simulink model "auto_sync_scan_module"  (R2016b)
settings: Solver=FixedStepDiscrete  StartTime=0.0  StopTime=3  FixedStep=Ts  RelTol=1e-3
InitFcn:
  | Ts = 50e-6;
values from neighbouring files (symbols this model uses):
  ScanStartTime = 0.2    [SISO_MIMO_blocks_Batch100_r2016b.m]
undefined symbols (not defined in the file or in its folder): freq
libraries: powerlib x17, powerlib_meascontrol x2
settings Model: Creator=rtlab17  LastModifiedBy=rtlab17

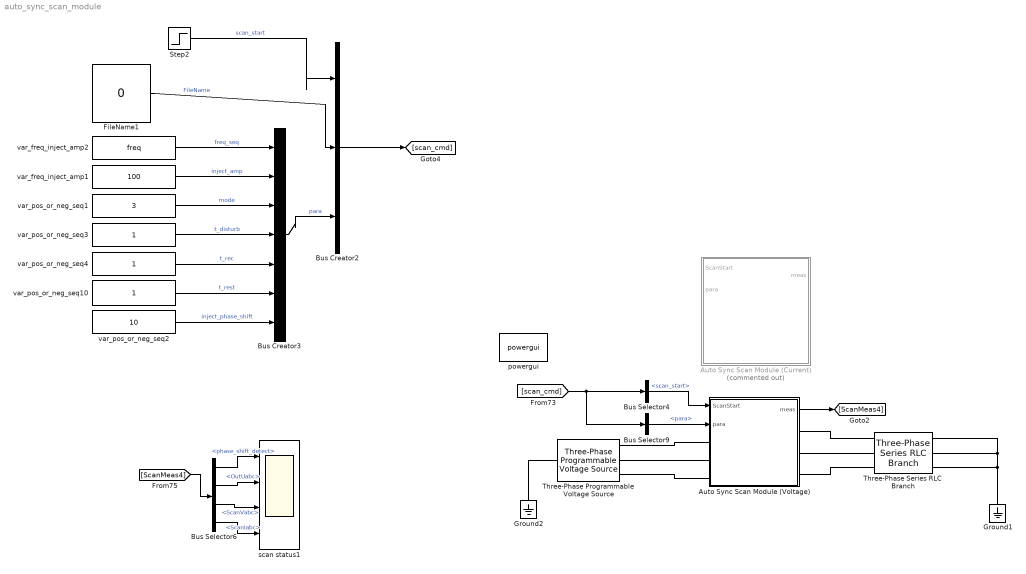
== system auto_sync_scan_module ==
  Auto Sync Scan Module (Current) : Subsystem  Commented=on  mask{var_gui_external=External, var_t_start=2, var_freq_seq=[1:350], var_inject_duration=1, var_record_duration=1, var_rest_duration=2, var_inject_amp=690*0.05, var_inject_mode=1, var_inject_phase_shift=0, var_ts=Ts}
      mask prompts: var_gui_external "Using"; var_t_start "Injection starting time (s)"; var_freq_seq "Frequency Sequence (Hz)"; var_inject_duration "Injection durtion (s)"; var_record_duration "Record duration (s), this set only output a recording signal"; var_rest_duration "Stable durtion (s)"; var_inject_amp "Injection magnitude. eg. 690*0.02"; var_inject_mode "Injection mode. eg 1 for Positive sequence, 2 for Negative, 3 for MIMO"; var_inject_phase_shift "Injection phase shift angle (deg). eg. if set 20 deg, disturb will injected when the phase angle 20deg of grid Uabc comes"; var_ts "Sample time"
      mask help:
      | |--------------Injection duration--------------|-----Stable duration------|
      |                      |-----Record duration-----|
      |
      | Record duration <= Inject duration
      |
      | Freq coupling implemented in this version
      mask init:
      | block = find_system(gcb,...
      |           'LookUnderMasks','on',...
      |           'FollowLinks','on','Name','In2');
      | % p=Simulink.Mask.get(gcb);
      | 
      | maskObj = Simulink.Mask.get(gcb);
      | [control, phandle] = maskObj.getDialogControl('para_group_gui_setting_zone');
      | 
      | switch var_gui_external
      |     case 1
      |         
      | %       if ~isempty(block)
      | % %         delete_block(block);
      | %         
      | %       end
      |       control.Visible = 'on';
      | 
      |       
      |       
      | %       p.getDialogControl('para_group_gui_setting_zone').Visible='on';
      |     case 2
      |         
      | %         if isempty(block)
      | % %             add_block('built-in/Inport',[gcb,'/In2']);
      | %         end
      |         
      |         control.Visible = 'off';
      | %         p.getDialogControl('para_group_gui_setting_zone').Visible='off';
      |     otherwise
      |         
      | end % switch
      | 
      | % disp(num2str(var_gui_external));
      mask Help:
      | by Yamin
      | v3(2024/11/28):
      | 1. fix: injection does not start when phase lag close to zero.
      | 2. refine the circuit connection topology.
      | 
      | v2(2024/5/17):
      | 1. add PLL phase alignment;
      | 2. Frequence sequence now can be specified by vector, elements could be random if you intend to do so.
      mask TypeOptions var_gui_external: GUI | External
      mask Display: text(0.3, 0.5, '电流源注入')
  Auto Sync Scan Module (Voltage) : Subsystem  mask{var_gui_external=External, var_t_start=2, var_freq_seq=[1:350], var_inject_duration=1, var_record_duration=1, var_rest_duration=2, var_inject_amp=690*0.05, var_inject_mode=1, var_inject_phase_shift=0, var_ts=Ts}
      mask prompts: var_gui_external "Using"; var_t_start "Injection starting time (s)"; var_freq_seq "Frequency Sequence (Hz)"; var_inject_duration "Injection durtion (s)"; var_record_duration "Record duration (s), this set only output a recording signal"; var_rest_duration "Stable durtion (s)"; var_inject_amp "Injection magnitude. eg. 690*0.02"; var_inject_mode "Injection mode. eg 1 for Positive sequence, 2 for Negative, 3 for MIMO"; var_inject_phase_shift "Injection phase shift angle (deg). eg. if set 20 deg, disturb will injected when the phase angle 20deg of grid Uabc comes"; var_ts "Sample time"
      mask help:
      | |--------------Injection duration--------------|-----Stable duration------|
      |                      |-----Record duration-----|
      |
      | Record duration <= Inject duration
      |
      | Freq coupling implemented in this version
      mask init: same as auto_sync_scan_module/Auto Sync Scan Module (Current)
      mask Help:
      | by Yamin
      | v3(2024/11/28):
      | 1. fix: injection does not start when phase lag close to zero.
      | 2. refine the circuit connection topology.
      | 
      | v2(2024/5/17):
      | 1. add PLL phase alignment;
      | 2. Frequence sequence now can be specified by vector, elements could be random if you intend to do so.
      mask TypeOptions var_gui_external: GUI | External
      mask Display: text(0.3, 0.5, '电压源注入')
  Bus Creator2 : BusCreator  Inputs=3
  Bus Creator3 : BusCreator  Inputs=7
  Bus Selector4 : BusSelector  OutputSignals=scan_start
  Bus Selector6 : BusSelector  OutputSignals=phase_shift_detect,OutUabc,ScanVabc,ScanIabc
  Bus Selector9 : BusSelector  OutputSignals=para
  FileName1 : Constant  Value=0
  Ground1 : powerlib/Elements/Ground  LConnTagsString=a
  Ground2 : powerlib/Elements/Ground  LConnTagsString=a
  Step2 : Step  Time=ScanStartTime  SampleTime=0
  Three-Phase Programmable Voltage Source : powerlib/Electrical Sources/Three-Phase Programmable Voltage Source  PositiveSequence="[230e3  0 50]"  VariationEntity=None  VariationType=Table of time-amplitude pairs  VariationTypeAlt=Step  VariationStep=0.5  VariationRate=10  VariationMagnitude=0.3  VariationFrequency=2  VariationTiming=[1 2]  VariationPhaseA=off  Amplitudes=[1 0.8 1.2 1.0]  TimeValues=[0 0.1 0.15 0.2]  HarmonicGeneration=off  HarmonicA=[3 0.2 -25 0]  HarmonicB=[2 0.15 35 2]  Timing="[0.05  3]"  BusType=PV  Pref=1100e6  Qref=0  Qmin=-inf  Qmax=inf
  Three-Phase Series RLC Branch : powerlib/Elements/Three-Phase Series RLC Branch  LConnTagsString=A|B|C  RConnTagsString=A|B|C  BranchType=RL  Resistance=1  Inductance=0.1  Capacitance=1e-6  Measurements=None
  powergui : powerlib/powergui  Priority=1  SimulationMode=Discrete  SolverType=Tustin/Backward Euler (TBE)  SampleTime=Ts  frequency=60  SPID=off  DisableSnubberDevices=off  DisableRonSwitches=off  DisableVfSwitches=off  SwTol=0  DisplayEquations=off  Interpol=off  ExternalGateDelay=off  methode=off  Ts=10  FunctionMessages=off  echomessages=off  HookPort=off  EnableUseOfTLC=off  x0status=blocks  frequencyindice=50  Pbase=100e6  ErrMax=1e-4  Iterations=50  UnitsV=kV  UnitsW=MW  buscounter=0  RestoreLinks=warning  ResistiveCurrentMeasurement=off  Frange=[0:2:500]  Ylog=off  Xlog=on  ShowGrid=off  save=off  variable=ZData  structure=0  ZoomFFT=off  StartTime=0.0  cycles=1  DisplayStyle=1  fundamental=60  FreqAxis=off  MaxFrequency=1000  frequencyindicesteady=1  RmsSteady=1  display=off
  scan status1 : Scope  NumInputPorts=4
  var_freq_inject_amp1 : Constant  Value=100
  var_freq_inject_amp2 : Constant  Value=freq
  var_pos_or_neg_seq1 : Constant  Value=3
  var_pos_or_neg_seq10 : Constant
  var_pos_or_neg_seq2 : Constant  Value=10
  var_pos_or_neg_seq3 : Constant
  var_pos_or_neg_seq4 : Constant
  wires:
  FileName1/1 -> Bus Creator2/2  "FileName"
  Step2/1 -> Bus Creator2/1  "scan_start"
  Bus Creator3/1 -> Bus Creator2/3  "para"
  var_freq_inject_amp1/1 -> Bus Creator3/2  "inject_amp"
  var_pos_or_neg_seq1/1 -> Bus Creator3/3  "mode"
  var_pos_or_neg_seq3/1 -> Bus Creator3/4  "t_disturb"
  var_pos_or_neg_seq4/1 -> Bus Creator3/5  "t_rec"
  var_pos_or_neg_seq10/1 -> Bus Creator3/6  "t_rest"
  var_freq_inject_amp2/1 -> Bus Creator3/1  "freq_seq"
  var_pos_or_neg_seq2/1 -> Bus Creator3/7  "inject_phase_shift"
  Bus Creator2/1 -> [scan_cmd]
  [ScanMeas4] -> Bus Selector6/1
  Bus Selector6/1 -> scan status1/1  "<phase_shift_detect>"
  Bus Selector6/2 -> scan status1/2  "<OutUabc>"
  Bus Selector4/1 -> Auto Sync Scan Module (Voltage)/1(ScanStart)  "<scan_start>"
  Bus Selector9/1 -> Auto Sync Scan Module (Voltage)/2(para)  "<para>"
  [scan_cmd] -> Bus Selector9/1, Bus Selector4/1
  Auto Sync Scan Module (Voltage)/1(meas) -> [ScanMeas4]
  Bus Selector6/3 -> scan status1/3  "<ScanVabc>"
  Bus Selector6/4 -> scan status1/4  "<ScanIabc>"
  connections:
  Ground2/LConn1 -- Three-Phase Programmable Voltage Source/LConn1
  Ground1/LConn1 -- Three-Phase Series RLC Branch/RConn3 -- Three-Phase Series RLC Branch/RConn1 -- Three-Phase Series RLC Branch/RConn2
  Auto Sync Scan Module (Voltage)/LConn2 -- Three-Phase Programmable Voltage Source/RConn2
  Auto Sync Scan Module (Voltage)/LConn3 -- Three-Phase Programmable Voltage Source/RConn3
  Auto Sync Scan Module (Voltage)/LConn1 -- Three-Phase Programmable Voltage Source/RConn1
  Auto Sync Scan Module (Voltage)/RConn1 -- Three-Phase Series RLC Branch/LConn1
  Auto Sync Scan Module (Voltage)/RConn2 -- Three-Phase Series RLC Branch/LConn2
  Auto Sync Scan Module (Voltage)/RConn3 -- Three-Phase Series RLC Branch/LConn3

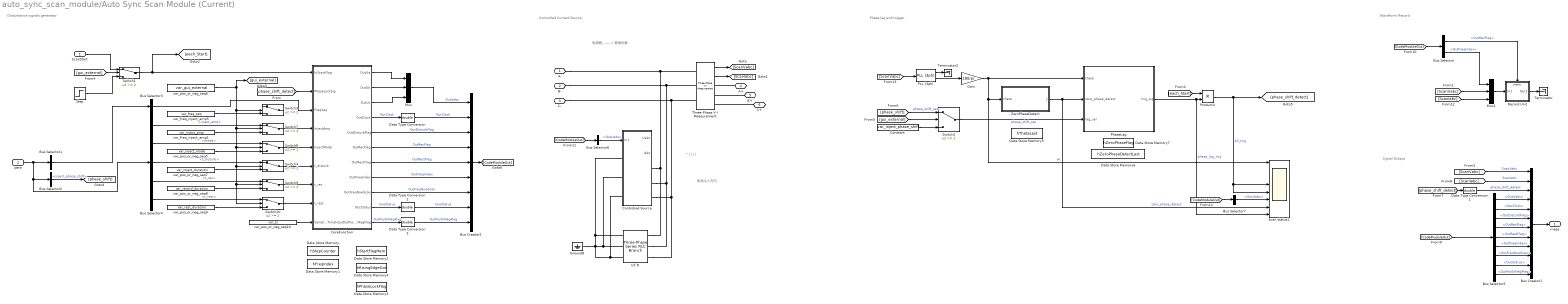
== system auto_sync_scan_module/Auto Sync Scan Module (Current) ==
  note: Disturbance signals generator
  note: Phase lag and trigger
  note: Waveform Record
  note: Signal Output
  note: 电流注入方向
  note: ^
      | |
      | |
      | |
      | |
  note: Controlled Current Source
  note: 电源侧 ------> 被测对象
  ScanStart : Inport
  para : Inport  Port=2
  Bus Creator1 : BusCreator  Inputs=12
  Bus Creator2 : BusCreator  Inputs=9
  Bus Selector : BusSelector  OutputSignals=OutRecFlag,OutFreqIndex
  Bus Selector1 : BusSelector  OutputSignals=freq_seq,inject_amp,mode,t_disturb,t_rec,t_rest  OutputAsBus=on
  Bus Selector2 : BusSelector  OutputSignals=inject_phase_shift
  Bus Selector3 : BusSelector  OutputSignals=freq_seq  OutputAsBus=on
  Bus Selector4 : BusSelector  OutputSignals=inject_amp,mode,t_disturb,t_rec,t_rest
  Bus Selector5 : BusSelector  OutputSignals=OutUabc,OutClock,OutDisturbFlag,OutRecFlag,OutRestFlag,OutFreqIndex,OutFreqNowScan,OutStatus,OutPosOrNegFlag
  Bus Selector6 : BusSelector  OutputSignals=OutUabc
  Bus Selector7 : BusSelector  OutputSignals=OutUabc
  Constant : Constant  Value=var_inject_phase_shift
  Controlled Source : Subsystem
  CoreFunction : MATLAB Function  TreatAsAtomicUnit=on  SystemSampleTime=var_ts
  Data Store Memory : DataStoreMemory  DataStoreName=hStepCounter  ReadBeforeWriteMsg=warning  WriteAfterWriteMsg=warning  WriteAfterReadMsg=warning  ShowAdditionalParam=off  OutDataTypeStr=int32
  Data Store Memory1 : DataStoreMemory  DataStoreName=hFreqIndex  ReadBeforeWriteMsg=warning  WriteAfterWriteMsg=warning  WriteAfterReadMsg=warning  ShowAdditionalParam=off  OutDataTypeStr=double
  Data Store Memory2 : DataStoreMemory  DataStoreName=hStartFlagMem  ReadBeforeWriteMsg=warning  WriteAfterWriteMsg=warning  WriteAfterReadMsg=warning  ShowAdditionalParam=off  OutDataTypeStr=int32
  Data Store Memory3 : DataStoreMemory  DataStoreName=hPhaseLockFlag  ReadBeforeWriteMsg=warning  WriteAfterWriteMsg=warning  WriteAfterReadMsg=warning  ShowAdditionalParam=off  OutDataTypeStr=double
  Data Store Memory4 : DataStoreMemory  DataStoreName=hRisingEdgeGot  ReadBeforeWriteMsg=warning  WriteAfterWriteMsg=warning  WriteAfterReadMsg=warning  ShowAdditionalParam=off  OutDataTypeStr=double
  Data Store Memory5 : DataStoreMemory  DataStoreName=hThetaLast  ReadBeforeWriteMsg=warning  WriteAfterWriteMsg=warning  WriteAfterReadMsg=warning  ShowAdditionalParam=off  OutDataTypeStr=double
  Data Store Memory6 : DataStoreMemory  DataStoreName=hZeroPhaseDetectLast  ReadBeforeWriteMsg=warning  WriteAfterWriteMsg=warning  WriteAfterReadMsg=warning  ShowAdditionalParam=off  OutDataTypeStr=double
  Data Store Memory7 : DataStoreMemory  DataStoreName=hZeroPhaseFlag  ReadBeforeWriteMsg=warning  WriteAfterWriteMsg=warning  WriteAfterReadMsg=warning  ShowAdditionalParam=off  OutDataTypeStr=double
  Data Type Conversion{,1..3} (4 alike) : DataTypeConversion  OutDataTypeStr=double
  Gain : Gain  Gain=180/pi
  Ground8 : powerlib/Elements/Ground  LConnTagsString=a
  Inf R : powerlib/Elements/Three-Phase Series RLC Branch  LConnTagsString=A|B|C  RConnTagsString=A|B|C  BranchType=R  Resistance=1e6  Inductance=4.57186*sin(deg2rad(85.2))/(100*pi)  Capacitance=1e-6  Measurements=None
  Mux : Mux  Inputs=3
  Mux1 : Mux  Inputs=3
  PLL (3ph) : powerlib_meascontrol/PLL/PLL (3ph)  Fmin=45  Par_Init=[0, 50]  ParK=[180, 3200, 1]  TcD=1e-4  MaxRateChangeFreq=12  FilterCutOffFreq=25  Ts=var_ts  AGC=on
  PhaseLag : MATLAB Function  TreatAsAtomicUnit=on
  Product4 : Product
  Record Unit : Subsystem
  Step : Step  Time=var_t_start  SampleTime=0
  Switch{1..2,4,7..10} (7 alike) : Switch  Threshold=2
  Switch3 : Switch  Threshold=2  AllowDiffInputSizes=on
  Terminator : Terminator
  Terminator2 : Terminator
  Three-Phase V-I Measurement : powerlib/Measurements/Three-Phase V-I Measurement  VoltageMeasurement=phase-to-ground  SetLabelV=off  LabelV=Vabc  Vpu=off  VpuLL=off  CurrentMeasurement=yes  SetLabelI=off  LabelI=Iabc  Ipu=off  Pbase=100e6  Vbase=500e3  OutputType=Complex  PhasorSimulation=off  PSBequivalent=0
  ZeroPhaseDetect : MATLAB Function  TreatAsAtomicUnit=on
  scan status1 : Scope  NumInputPorts=8
  var_freq_inject_amp1 : Constant  Value=var_inject_amp
  var_freq_inject_amp5 : Constant  Value=var_freq_seq
  var_pos_or_neg_seq10 : Constant  Value=var_ts
  var_pos_or_neg_seq5 : Constant  Value=var_inject_mode
  var_pos_or_neg_seq6 : Constant  Value=var_gui_external
  var_pos_or_neg_seq7 : Constant  Value=var_inject_duration
  var_pos_or_neg_seq8 : Constant  Value=var_record_duration
  var_pos_or_neg_seq9 : Constant  Value=var_rest_duration
  A- : PMIOPort  Port=1  Side=Left
  B- : PMIOPort  Port=2  Side=Left
  C- : PMIOPort  Port=3  Side=Left
  A+ : PMIOPort  Port=4  Side=Right
  B+ : PMIOPort  Port=5  Side=Right
  C+ : PMIOPort  Port=6  Side=Right
  meas : Outport
  wires:
  CoreFunction/9(OutFreqNowScan) -> Bus Creator2/7  "OutFreqNowScan"
  Bus Selector/1 -> Record Unit/Enable  "<OutRecFlag>"
  Bus Selector1/1 -> Bus Selector3/1
  var_pos_or_neg_seq10/1 -> CoreFunction/9(SampleTimeInput)
  var_pos_or_neg_seq6/1 -> Switch3/2, Switch7/2, Switch8/2, Switch4/2, Switch9/2, Switch10/2, [gui_external]
  CoreFunction/8(OutFreqIndex) -> Bus Creator2/6  "OutFreqIndex"
  CoreFunction/7(OutRestFlag) -> Bus Creator2/5  "OutRestFlag"
  CoreFunction/5(OutDisturbFlag) -> Bus Creator2/3  "OutDisturbFlag"
  CoreFunction/6(OutRecFlag) -> Bus Creator2/4  "OutRecFlag"
  Data Type Conversion2/1 -> Bus Creator2/8  "OutStatus"
  Data Type Conversion/1 -> Bus Creator2/2  "OutClock"
  Data Type Conversion3/1 -> Bus Creator2/9  "OutPosOrNegFlag"
  Mux/1 -> Bus Creator2/1  "OutUabc"
  CoreFunction/1(OutUa) -> Mux/1
  CoreFunction/3(OutUc) -> Mux/3
  CoreFunction/2(OutUb) -> Mux/2
  Switch7/1 -> CoreFunction/4(InjectAmp)
  Switch8/1 -> CoreFunction/5(InjectMode)
  Switch4/1 -> CoreFunction/6(t_disturb)
  Switch9/1 -> CoreFunction/7(t_rec)
  Switch10/1 -> CoreFunction/8(t_rest)
  var_pos_or_neg_seq9/1 -> Switch10/3
  var_pos_or_neg_seq8/1 -> Switch9/3
  var_pos_or_neg_seq7/1 -> Switch4/3
  var_pos_or_neg_seq5/1 -> Switch8/3
  var_freq_inject_amp1/1 -> Switch7/3
  var_freq_inject_amp5/1 -> Switch3/3
  Bus Selector4/1 -> Switch7/1  "<inject_amp>"
  Bus Selector4/4 -> Switch9/1  "<t_rec>"
  Bus Selector4/3 -> Switch4/1  "<t_disturb>"
  Bus Selector4/5 -> Switch10/1  "<t_rest>"
  Bus Selector4/2 -> Switch8/1  "<mode>"
  Bus Selector3/1 -> CoreFunction/3(FreqSeq)
  CoreFunction/11(OutPosOrNegFlag) -> Data Type Conversion3/1  "OutPosOrNegFlag"
  CoreFunction/10(OutStatus) -> Data Type Conversion2/1  "OutStatus"
  CoreFunction/4(OutClock) -> Data Type Conversion/1  "OutClock"
  Bus Selector/2 -> Mux1/1  "<OutFreqIndex>"
  Mux1/1 -> Record Unit/1(In1)
  Bus Creator2/1 -> [CodeModuleOut]
  PLL (3ph)/2 -> Gain/1
  Gain/1 -> scan status1/1, ZeroPhaseDetect/1(theta), PhaseLag/1(theta)  "wt"
  Constant/1 -> Switch2/3
  Product4/1 -> scan status1/5, scan status1/4, [phase_shift_detect]  "pll_trig"
  [each_Start] -> Product4/1
  Switch1/1 -> [each_Start], CoreFunction/1(InStartFlag)
  ScanStart/1 -> Switch1/1
  Step/1 -> Switch1/3
  Switch2/1 -> PhaseLag/3(lag_val)  "phase_shift_set"
  [gui_external] -> Switch2/2
  [gui_external] -> Switch1/2
  para/1 -> Bus Selector1/1, Bus Selector4/1, Bus Selector2/1
  Bus Selector2/1 -> [phase_shift]  "<inject_phase_shift>"
  [phase_shift] -> Switch2/1  "phase_shift_set"
  Bus Creator1/1 -> meas/1
  PLL (3ph)/1 -> Terminator2/1
  [phase_shift_detect] -> Data Type Conversion1/1
  Data Type Conversion1/1 -> Bus Creator1/3  "phase_shift_detect"
  [ScanVabc] -> Bus Creator1/1  "ScanVabc"
  [ScanIabc] -> Bus Creator1/2  "ScanIabc"
  Bus Selector5/3 -> Bus Creator1/6  "<OutDisturbFlag>"
  Bus Selector5/2 -> Bus Creator1/5  "<OutClock>"
  Bus Selector5/4 -> Bus Creator1/7  "<OutRecFlag>"
  Bus Selector5/1 -> Bus Creator1/4  "<OutUabc>"
  Bus Selector5/5 -> Bus Creator1/8  "<OutRestFlag>"
  Bus Selector5/6 -> Bus Creator1/9  "<OutFreqIndex>"
  Bus Selector5/7 -> Bus Creator1/10  "<OutFreqNowScan>"
  Bus Selector5/8 -> Bus Creator1/11  "<OutStatus>"
  Bus Selector5/9 -> Bus Creator1/12  "<OutPosOrNegFlag>"
  [CodeModuleOut] -> Bus Selector5/1
  Record Unit/1(Out1) -> Terminator/1
  [CodeModuleOut] -> Bus Selector/1
  ZeroPhaseDetect/1(y) -> scan status1/7, PhaseLag/2(zero_phase_detect)  "zero_phase_detect"
  PhaseLag/1(trig_sig) -> scan status1/8, Product4/2  "phase_lag_trig"
  [phase_shift_detect] -> CoreFunction/2(PhaseLockSig)
  [ScanVabc] -> Mux1/2
  [ScanIabc] -> Mux1/3
  [ScanVabc] -> PLL (3ph)/1
  [CodeModuleOut] -> Bus Selector7/1
  Bus Selector7/1 -> scan status1/6  "<OutUabc>"
  [CodeModuleOut] -> Bus Selector6/1
  Three-Phase V-I Measurement/2 -> [ScanIabc]
  Three-Phase V-I Measurement/1 -> [ScanVabc]
  Bus Selector6/1 -> Controlled Source/1(In1)  "<OutUabc>"
  connections:
  Controlled Source/RConn2 -- Inf R/LConn2 -- Three-Phase V-I Measurement/LConn2 -- B-/RConn1
  Inf R/LConn3 -- Controlled Source/RConn3 -- Three-Phase V-I Measurement/LConn3 -- C-/RConn1
  A-/RConn1 -- Three-Phase V-I Measurement/LConn1 -- Inf R/LConn1 -- Controlled Source/RConn1
  Controlled Source/LConn3 -- Inf R/RConn3 -- Ground8/LConn1 -- Inf R/RConn1 -- Controlled Source/LConn1 -- Inf R/RConn2 -- Controlled Source/LConn2
  C+/RConn1 -- Three-Phase V-I Measurement/RConn3
  B+/RConn1 -- Three-Phase V-I Measurement/RConn2
  A+/RConn1 -- Three-Phase V-I Measurement/RConn1

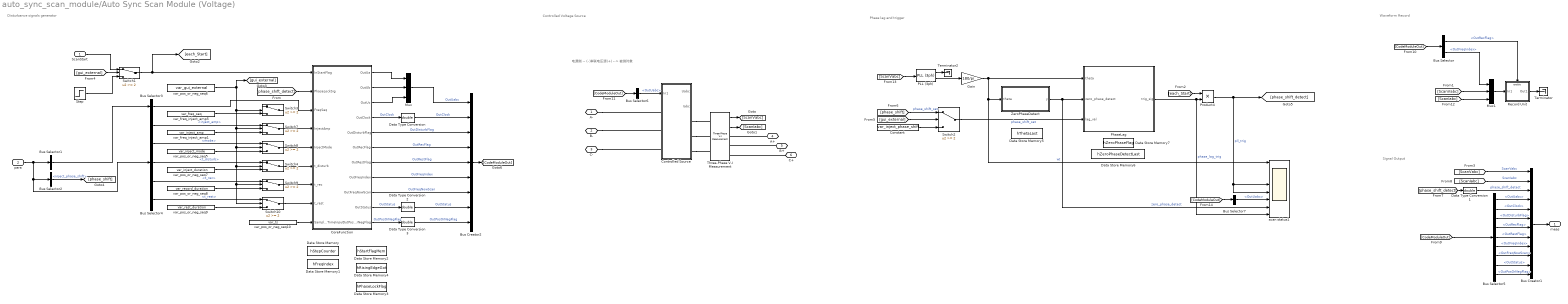
== system auto_sync_scan_module/Auto Sync Scan Module (Voltage) ==
  note: Signal Output
  note: Waveform Record
  note: Phase lag and trigger
  note: Disturbance signals generator
  note: Controlled Voltage Source
  note: 电源侧 -- (-)串联电压源(+) --> 被测对象
  ScanStart : Inport
  para : Inport  Port=2
  Bus Creator1 : BusCreator  Inputs=12
  Bus Creator2 : BusCreator  Inputs=9
  Bus Selector : BusSelector  OutputSignals=OutRecFlag,OutFreqIndex
  Bus Selector1 : BusSelector  OutputSignals=freq_seq,inject_amp,mode,t_disturb,t_rec,t_rest  OutputAsBus=on
  Bus Selector2 : BusSelector  OutputSignals=inject_phase_shift
  Bus Selector3 : BusSelector  OutputSignals=freq_seq  OutputAsBus=on
  Bus Selector4 : BusSelector  OutputSignals=inject_amp,mode,t_disturb,t_rec,t_rest
  Bus Selector5 : BusSelector  OutputSignals=OutUabc,OutClock,OutDisturbFlag,OutRecFlag,OutRestFlag,OutFreqIndex,OutFreqNowScan,OutStatus,OutPosOrNegFlag
  Bus Selector6 : BusSelector  OutputSignals=OutUabc
  Bus Selector7 : BusSelector  OutputSignals=OutUabc
  Constant : Constant  Value=var_inject_phase_shift
  Controlled Source : Subsystem
  CoreFunction : MATLAB Function  TreatAsAtomicUnit=on  SystemSampleTime=var_ts
  Data Store Memory : DataStoreMemory  DataStoreName=hStepCounter  ReadBeforeWriteMsg=warning  WriteAfterWriteMsg=warning  WriteAfterReadMsg=warning  ShowAdditionalParam=off  OutDataTypeStr=int32
  Data Store Memory1 : DataStoreMemory  DataStoreName=hFreqIndex  ReadBeforeWriteMsg=warning  WriteAfterWriteMsg=warning  WriteAfterReadMsg=warning  ShowAdditionalParam=off  OutDataTypeStr=double
  Data Store Memory2 : DataStoreMemory  DataStoreName=hStartFlagMem  ReadBeforeWriteMsg=warning  WriteAfterWriteMsg=warning  WriteAfterReadMsg=warning  ShowAdditionalParam=off  OutDataTypeStr=int32
  Data Store Memory3 : DataStoreMemory  DataStoreName=hPhaseLockFlag  ReadBeforeWriteMsg=warning  WriteAfterWriteMsg=warning  WriteAfterReadMsg=warning  ShowAdditionalParam=off  OutDataTypeStr=double
  Data Store Memory4 : DataStoreMemory  DataStoreName=hRisingEdgeGot  ReadBeforeWriteMsg=warning  WriteAfterWriteMsg=warning  WriteAfterReadMsg=warning  ShowAdditionalParam=off  OutDataTypeStr=double
  Data Store Memory5 : DataStoreMemory  DataStoreName=hThetaLast  ReadBeforeWriteMsg=warning  WriteAfterWriteMsg=warning  WriteAfterReadMsg=warning  ShowAdditionalParam=off  OutDataTypeStr=double
  Data Store Memory6 : DataStoreMemory  DataStoreName=hZeroPhaseDetectLast  ReadBeforeWriteMsg=warning  WriteAfterWriteMsg=warning  WriteAfterReadMsg=warning  ShowAdditionalParam=off  OutDataTypeStr=double
  Data Store Memory7 : DataStoreMemory  DataStoreName=hZeroPhaseFlag  ReadBeforeWriteMsg=warning  WriteAfterWriteMsg=warning  WriteAfterReadMsg=warning  ShowAdditionalParam=off  OutDataTypeStr=double
  Data Type Conversion{,1..3} (4 alike) : DataTypeConversion  OutDataTypeStr=double
  Gain : Gain  Gain=180/pi
  Mux : Mux  Inputs=3
  Mux1 : Mux  Inputs=3
  PLL (3ph) : powerlib_meascontrol/PLL/PLL (3ph)  Fmin=45  Par_Init=[0, 50]  ParK=[180, 3200, 1]  TcD=1e-4  MaxRateChangeFreq=12  FilterCutOffFreq=25  Ts=var_ts  AGC=on
  PhaseLag : MATLAB Function  TreatAsAtomicUnit=on
  Product4 : Product
  Record Unit : Subsystem
  Step : Step  Time=var_t_start  SampleTime=0
  Switch{1..2,4,7..10} (7 alike) : Switch  Threshold=2
  Switch3 : Switch  Threshold=2  AllowDiffInputSizes=on
  Terminator : Terminator
  Terminator2 : Terminator
  Three-Phase V-I Measurement : powerlib/Measurements/Three-Phase V-I Measurement  VoltageMeasurement=phase-to-ground  SetLabelV=off  LabelV=Vabc  Vpu=off  VpuLL=off  CurrentMeasurement=yes  SetLabelI=off  LabelI=Iabc  Ipu=off  Pbase=100e6  Vbase=500e3  OutputType=Complex  PhasorSimulation=off  PSBequivalent=0
  ZeroPhaseDetect : MATLAB Function  TreatAsAtomicUnit=on
  scan status1 : Scope  NumInputPorts=8
  var_freq_inject_amp1 : Constant  Value=var_inject_amp
  var_freq_inject_amp5 : Constant  Value=var_freq_seq
  var_pos_or_neg_seq10 : Constant  Value=var_ts
  var_pos_or_neg_seq5 : Constant  Value=var_inject_mode
  var_pos_or_neg_seq6 : Constant  Value=var_gui_external
  var_pos_or_neg_seq7 : Constant  Value=var_inject_duration
  var_pos_or_neg_seq8 : Constant  Value=var_record_duration
  var_pos_or_neg_seq9 : Constant  Value=var_rest_duration
  A- : PMIOPort  Port=1  Side=Left
  B- : PMIOPort  Port=2  Side=Left
  C- : PMIOPort  Port=3  Side=Left
  A+ : PMIOPort  Port=4  Side=Right
  B+ : PMIOPort  Port=5  Side=Right
  C+ : PMIOPort  Port=6  Side=Right
  meas : Outport
  wires:
  Bus Selector7/1 -> scan status1/6  "<OutUabc>"
  [CodeModuleOut] -> Bus Selector7/1
  [ScanVabc] -> PLL (3ph)/1
  [ScanIabc] -> Mux1/3
  [ScanVabc] -> Mux1/2
  [phase_shift_detect] -> CoreFunction/2(PhaseLockSig)
  PhaseLag/1(trig_sig) -> Product4/2, scan status1/8  "phase_lag_trig"
  ZeroPhaseDetect/1(y) -> PhaseLag/2(zero_phase_detect), scan status1/7  "zero_phase_detect"
  [CodeModuleOut] -> Bus Selector6/1
  [CodeModuleOut] -> Bus Selector/1
  Record Unit/1(Out1) -> Terminator/1
  [CodeModuleOut] -> Bus Selector5/1
  Bus Selector5/9 -> Bus Creator1/12  "<OutPosOrNegFlag>"
  Bus Selector5/8 -> Bus Creator1/11  "<OutStatus>"
  Bus Selector5/7 -> Bus Creator1/10  "<OutFreqNowScan>"
  Bus Selector5/6 -> Bus Creator1/9  "<OutFreqIndex>"
  Bus Selector5/5 -> Bus Creator1/8  "<OutRestFlag>"
  Bus Selector5/1 -> Bus Creator1/4  "<OutUabc>"
  Bus Selector5/4 -> Bus Creator1/7  "<OutRecFlag>"
  Bus Selector5/2 -> Bus Creator1/5  "<OutClock>"
  Bus Selector5/3 -> Bus Creator1/6  "<OutDisturbFlag>"
  [ScanIabc] -> Bus Creator1/2  "ScanIabc"
  [ScanVabc] -> Bus Creator1/1  "ScanVabc"
  Data Type Conversion1/1 -> Bus Creator1/3  "phase_shift_detect"
  [phase_shift_detect] -> Data Type Conversion1/1
  PLL (3ph)/1 -> Terminator2/1
  Bus Creator1/1 -> meas/1
  [phase_shift] -> Switch2/1  "phase_shift_set"
  Bus Selector2/1 -> [phase_shift]  "<inject_phase_shift>"
  para/1 -> Bus Selector2/1, Bus Selector4/1, Bus Selector1/1
  [gui_external] -> Switch1/2
  [gui_external] -> Switch2/2
  Switch2/1 -> PhaseLag/3(lag_val)  "phase_shift_set"
  Three-Phase V-I Measurement/2 -> [ScanIabc]
  Step/1 -> Switch1/3
  ScanStart/1 -> Switch1/1
  Switch1/1 -> CoreFunction/1(InStartFlag), [each_Start]
  [each_Start] -> Product4/1
  Product4/1 -> [phase_shift_detect], scan status1/4, scan status1/5  "pll_trig"
  Constant/1 -> Switch2/3
  Gain/1 -> PhaseLag/1(theta), ZeroPhaseDetect/1(theta), scan status1/1  "wt"
  PLL (3ph)/2 -> Gain/1
  Three-Phase V-I Measurement/1 -> [ScanVabc]
  Bus Creator2/1 -> [CodeModuleOut]
  Bus Selector6/1 -> Controlled Source/1(In1)  "<OutUabc>"
  Mux1/1 -> Record Unit/1(In1)
  Bus Selector/2 -> Mux1/1  "<OutFreqIndex>"
  CoreFunction/4(OutClock) -> Data Type Conversion/1  "OutClock"
  CoreFunction/10(OutStatus) -> Data Type Conversion2/1  "OutStatus"
  CoreFunction/11(OutPosOrNegFlag) -> Data Type Conversion3/1  "OutPosOrNegFlag"
  Bus Selector3/1 -> CoreFunction/3(FreqSeq)
  Bus Selector4/2 -> Switch8/1  "<mode>"
  Bus Selector4/5 -> Switch10/1  "<t_rest>"
  Bus Selector4/3 -> Switch4/1  "<t_disturb>"
  Bus Selector4/4 -> Switch9/1  "<t_rec>"
  Bus Selector4/1 -> Switch7/1  "<inject_amp>"
  var_freq_inject_amp5/1 -> Switch3/3
  var_freq_inject_amp1/1 -> Switch7/3
  var_pos_or_neg_seq5/1 -> Switch8/3
  var_pos_or_neg_seq7/1 -> Switch4/3
  var_pos_or_neg_seq8/1 -> Switch9/3
  var_pos_or_neg_seq9/1 -> Switch10/3
  Switch10/1 -> CoreFunction/8(t_rest)
  Switch9/1 -> CoreFunction/7(t_rec)
  Switch4/1 -> CoreFunction/6(t_disturb)
  Switch8/1 -> CoreFunction/5(InjectMode)
  Switch7/1 -> CoreFunction/4(InjectAmp)
  CoreFunction/2(OutUb) -> Mux/2
  CoreFunction/3(OutUc) -> Mux/3
  CoreFunction/1(OutUa) -> Mux/1
  Mux/1 -> Bus Creator2/1  "OutUabc"
  Data Type Conversion3/1 -> Bus Creator2/9  "OutPosOrNegFlag"
  Data Type Conversion/1 -> Bus Creator2/2  "OutClock"
  Data Type Conversion2/1 -> Bus Creator2/8  "OutStatus"
  CoreFunction/6(OutRecFlag) -> Bus Creator2/4  "OutRecFlag"
  CoreFunction/5(OutDisturbFlag) -> Bus Creator2/3  "OutDisturbFlag"
  CoreFunction/7(OutRestFlag) -> Bus Creator2/5  "OutRestFlag"
  CoreFunction/8(OutFreqIndex) -> Bus Creator2/6  "OutFreqIndex"
  var_pos_or_neg_seq6/1 -> [gui_external], Switch10/2, Switch9/2, Switch4/2, Switch8/2, Switch7/2, Switch3/2
  var_pos_or_neg_seq10/1 -> CoreFunction/9(SampleTimeInput)
  Bus Selector1/1 -> Bus Selector3/1
  Bus Selector/1 -> Record Unit/Enable  "<OutRecFlag>"
  CoreFunction/9(OutFreqNowScan) -> Bus Creator2/7  "OutFreqNowScan"
  connections:
  C+/RConn1 -- Three-Phase V-I Measurement/RConn3
  B+/RConn1 -- Three-Phase V-I Measurement/RConn2
  A+/RConn1 -- Three-Phase V-I Measurement/RConn1
  Controlled Source/RConn2 -- Three-Phase V-I Measurement/LConn2
  Controlled Source/RConn3 -- Three-Phase V-I Measurement/LConn3
  Controlled Source/RConn1 -- Three-Phase V-I Measurement/LConn1
  C-/RConn1 -- Controlled Source/LConn3
  B-/RConn1 -- Controlled Source/LConn2
  A-/RConn1 -- Controlled Source/LConn1

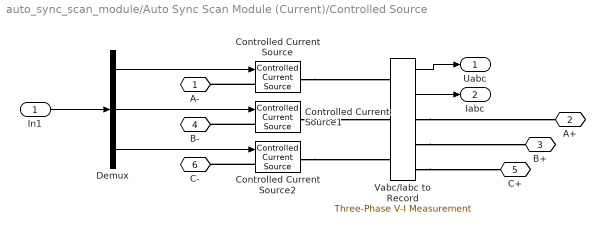
== system auto_sync_scan_module/Auto Sync Scan Module (Current)/Controlled Source ==
  In1 : Inport
  Controlled Current Source : powerlib/Electrical Sources/Controlled Current Source  Initialize=on  Source_Type=AC  Amplitude=0  Phase=0  Frequency=0  Measurements=None
  Controlled Current Source1 : powerlib/Electrical Sources/Controlled Current Source  Initialize=on  Source_Type=AC  Amplitude=0  Phase=0  Frequency=0  Measurements=None
  Controlled Current Source2 : powerlib/Electrical Sources/Controlled Current Source  Initialize=on  Source_Type=AC  Amplitude=0  Phase=0  Frequency=0  Measurements=None
  Demux : Demux  Outputs=3
  Vabc/Iabc to Record : powerlib/Measurements/Three-Phase V-I Measurement  VoltageMeasurement=phase-to-ground  SetLabelV=off  LabelV=ScanVabc  Vpu=off  VpuLL=off  CurrentMeasurement=yes  SetLabelI=off  LabelI=ScanIabc  Ipu=off  Pbase=100e6  Vbase=500e3  OutputType=Complex  PhasorSimulation=off  PSBequivalent=0
  A- : PMIOPort  Port=1  Side=Left
  A+ : PMIOPort  Port=2  Side=Right
  B+ : PMIOPort  Port=3  Side=Right
  B- : PMIOPort  Port=4  Side=Left
  C+ : PMIOPort  Port=5  Side=Right
  C- : PMIOPort  Port=6  Side=Left
  Uabc : Outport
  Iabc : Outport  Port=2
  wires:
  Demux/3 -> Controlled Current Source2/1
  Demux/2 -> Controlled Current Source1/1
  Demux/1 -> Controlled Current Source/1
  In1/1 -> Demux/1
  Vabc/Iabc to Record/1 -> Uabc/1
  Vabc/Iabc to Record/2 -> Iabc/1
  connections:
  Vabc/Iabc to Record/RConn1 -- A+/RConn1
  Controlled Current Source/RConn1 -- Vabc/Iabc to Record/LConn1
  Controlled Current Source1/RConn1 -- Vabc/Iabc to Record/LConn2
  Controlled Current Source2/RConn1 -- Vabc/Iabc to Record/LConn3
  Vabc/Iabc to Record/RConn3 -- C+/RConn1
  Controlled Current Source/LConn1 -- A-/RConn1
  Controlled Current Source1/LConn1 -- B-/RConn1
  Vabc/Iabc to Record/RConn2 -- B+/RConn1
  Controlled Current Source2/LConn1 -- C-/RConn1

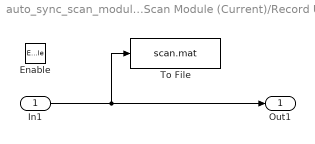
== system auto_sync_scan_module/Auto Sync Scan Module (Current)/Record Unit ==
  In1 : Inport
  Enable : EnablePort
  To File : ToFile  Filename=scan.mat  MatrixName=scan  SampleTime=var_ts
  Out1 : Outport
  wires:
  In1/1 -> Out1/1, To File/1

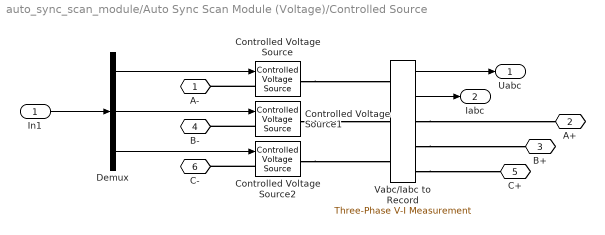
== system auto_sync_scan_module/Auto Sync Scan Module (Voltage)/Controlled Source ==
  In1 : Inport
  Controlled Voltage Source : powerlib/Electrical Sources/Controlled Voltage Source  Initialize=on  Source_Type=AC  Amplitude=0  Phase=0  Frequency=0  Measurements=None
  Controlled Voltage Source1 : powerlib/Electrical Sources/Controlled Voltage Source  Initialize=on  Source_Type=AC  Amplitude=0  Phase=0  Frequency=0  Measurements=None
  Controlled Voltage Source2 : powerlib/Electrical Sources/Controlled Voltage Source  Initialize=on  Source_Type=AC  Amplitude=0  Phase=0  Frequency=0  Measurements=None
  Demux : Demux  Outputs=3
  Vabc/Iabc to Record : powerlib/Measurements/Three-Phase V-I Measurement  VoltageMeasurement=phase-to-ground  SetLabelV=off  LabelV=ScanVabc  Vpu=off  VpuLL=off  CurrentMeasurement=yes  SetLabelI=off  LabelI=ScanIabc  Ipu=off  Pbase=100e6  Vbase=500e3  OutputType=Complex  PhasorSimulation=off  PSBequivalent=0
  A- : PMIOPort  Port=1  Side=Left
  A+ : PMIOPort  Port=2  Side=Right
  B+ : PMIOPort  Port=3  Side=Right
  B- : PMIOPort  Port=4  Side=Left
  C+ : PMIOPort  Port=5  Side=Right
  C- : PMIOPort  Port=6  Side=Left
  Uabc : Outport
  Iabc : Outport  Port=2
  wires:
  Demux/3 -> Controlled Voltage Source2/1
  Demux/2 -> Controlled Voltage Source1/1
  Demux/1 -> Controlled Voltage Source/1
  In1/1 -> Demux/1
  Vabc/Iabc to Record/1 -> Uabc/1
  Vabc/Iabc to Record/2 -> Iabc/1
  connections:
  Vabc/Iabc to Record/RConn1 -- A+/RConn1
  Controlled Voltage Source/RConn1 -- Vabc/Iabc to Record/LConn1
  Controlled Voltage Source1/RConn1 -- Vabc/Iabc to Record/LConn2
  Controlled Voltage Source2/RConn1 -- Vabc/Iabc to Record/LConn3
  Vabc/Iabc to Record/RConn3 -- C+/RConn1
  Controlled Voltage Source/LConn1 -- A-/RConn1
  Controlled Voltage Source1/LConn1 -- B-/RConn1
  Vabc/Iabc to Record/RConn2 -- B+/RConn1
  Controlled Voltage Source2/LConn1 -- C-/RConn1

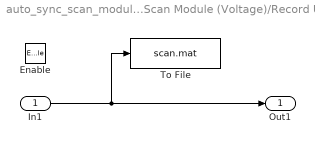
== system auto_sync_scan_module/Auto Sync Scan Module (Voltage)/Record Unit ==
  In1 : Inport
  Enable : EnablePort
  To File : ToFile  Filename=scan.mat  MatrixName=scan  SampleTime=var_ts
  Out1 : Outport
  wires:
  In1/1 -> To File/1, Out1/1

== matlab function auto_sync_scan_module/Auto Sync Scan Module (Current)/CoreFunction ==
  data: InStartFlag input; PhaseLockSig input; FreqSeq input; OutUa output; InjectAmp input; InjectMode input; t_disturb input; t_rec input; t_rest input; OutUb output; OutUc output; OutClock output; OutDisturbFlag output; OutRecFlag output; OutRestFlag output; OutFreqIndex output; OutFreqNowScan output; OutStatus output; OutPosOrNegFlag output; hStepCounter data_store_memory; hFreqIndex data_store_memory; hStartFlagMem data_store_memory; hPhaseLockFlag data_store_memory; SampleTimeInput input; hRisingEdgeGot data_store_memory
function [OutUa, OutUb, OutUc, ...
    OutClock, OutDisturbFlag, OutRecFlag, OutRestFlag, ...
    OutFreqIndex, OutFreqNowScan, OutStatus, OutPosOrNegFlag] = ...
    fcn(InStartFlag, PhaseLockSig, FreqSeq, InjectAmp, InjectMode, ...
    t_disturb, t_rec, t_rest, SampleTimeInput)
% InjectMode = 1, Positive sequence
% InjectMode = 2, Negative sequence
% InjectMode = 3, Positive et Negative simutaneously

global hStepCounter;
global hFreqIndex; 
global hStartFlagMem;
global hPhaseLockFlag;
global hRisingEdgeGot; % record a rising-edge get event, cleared untile all frequency are scanned.

this_freq = 0; %% only used for output
FreqSeqLength = length(FreqSeq);

SAMPLE_TIME = SampleTimeInput;
SAMPLE_FREQ = 1/SAMPLE_TIME;

T_DISTURB	= t_disturb * SAMPLE_FREQ;
T_REC 		= t_rec * SAMPLE_FREQ;
T_REST 		= t_rest * SAMPLE_FREQ;

clock_t		= 0;
start_flag	= 0;
status_code	= 0;
ua			= 0; 
ub			= 0; 
uc			= 0;
omega		= 0;
disturb_flag = 0;
rec_flag    = 0;
rest_flag   = 0;

if hPhaseLockFlag == 0 && PhaseLockSig == 1  % Phase-lock event catch, reset by every scan step
    hPhaseLockFlag = 1;
end


start_flag = InStartFlag;
if (start_flag >= 1 && hStartFlagMem == 0) % rising-edge event catch
	hRisingEdgeGot = 1;
	hFreqIndex = 1;
end

if (start_flag >= 1 && hRisingEdgeGot == 1) % once triggerd, loop until all frequences are scanned
	if (hFreqIndex >=1 && hFreqIndex <= FreqSeqLength && hPhaseLockFlag == 1)
		status_code = 1;
		if (hStepCounter <= (T_DISTURB - T_REC))
			disturb_flag = 1;
			rec_flag = 0;
			rest_flag = 0;
			hStepCounter = hStepCounter + 1;
        elseif ((hStepCounter > (T_DISTURB - T_REC)) && (hStepCounter <= T_DISTURB) && hPhaseLockFlag == 1)
			disturb_flag = 1;
			rec_flag = 1;
			rest_flag = 0;
			hStepCounter = hStepCounter + 1;
        elseif ((hStepCounter > T_DISTURB) && hStepCounter <= (T_DISTURB + T_REST) && hPhaseLockFlag == 1)
			disturb_flag = 0;
			rec_flag = 0;
			rest_flag = 1;
			hStepCounter = hStepCounter + 1;
        else
			hStepCounter = int32(0);
			hFreqIndex = hFreqIndex + 1;
			ua = 0; ub = 0; uc = 0;
            hPhaseLockFlag = 0;
        end

		if (disturb_flag == 1) 
            this_freq = FreqSeq(hFreqIndex); % only used for output port 
			clock_t = double(hStepCounter) * SAMPLE_TIME;
			omega = 2.0 * FreqSeq(hFreqIndex) * pi;
            
			if (InjectMode == 1)
				ua = InjectAmp * sin(omega * clock_t);
				ub = InjectAmp * sin(omega * clock_t - 2.0*pi/3.0);
				uc = InjectAmp * sin(omega * clock_t + 2.0*pi/3.0);
			
            elseif (InjectMode == 2)
				ua = InjectAmp * sin(omega * clock_t);
				ub = InjectAmp * sin(omega * clock_t + 2.0*pi/3.0);
				uc = InjectAmp * sin(omega * clock_t - 2.0*pi/3.0);
                
            elseif (InjectMode == 3)
                ua = InjectAmp * sin(omega * clock_t);
				ub = 0.5 * InjectAmp * sin(omega * clock_t + 2.0*pi/3.0) + ...
                     0.5 * InjectAmp * sin(omega * clock_t - 2.0*pi/3.0);
				uc = ub;
            else
                % other InjectMode to be write here.
            end
        end
	elseif hFreqIndex > FreqSeqLength
		status_code = 2;
		hRisingEdgeGot = 0;
		ua = 0; ub = 0; uc = 0;
	else
		ua = 0; ub = 0; uc = 0;
		status_code = 3;
	end

else % start_flag == 0 || hRisingEdgeGot == 0

	hFreqIndex = 1;

	status_code = 0;
	disturb_flag = 0;
	rec_flag = 0;
	rest_flag = 0;
	hStepCounter = int32(0);
	clock_t = double(hStepCounter) * SAMPLE_TIME;
	ua = 0; ub = 0; uc = 0;
end
	hStartFlagMem = int32(start_flag);  % record start_flag
	OutUa = ua;
	OutUb = ub;
	OutUc = uc;

	OutStatus = status_code;
	OutFreqIndex = hFreqIndex;
	OutFreqNowScan = this_freq;
	OutClock = clock_t;
	OutDisturbFlag = disturb_flag;
	OutRecFlag = rec_flag;
	OutRestFlag = rest_flag;
    OutPosOrNegFlag = InjectMode;
end

== matlab function auto_sync_scan_module/Auto Sync Scan Module (Current)/ZeroPhaseDetect ==
  data: theta input; y output; hThetaLast data_store_memory
function y = ZeroPhaseDetect(theta)
global hThetaLast;


if theta < hThetaLast
    zero_phase_detect = 1;
else
    zero_phase_detect = 0;
end
hThetaLast = theta;

y = zero_phase_detect;

== matlab function auto_sync_scan_module/Auto Sync Scan Module (Current)/PhaseLag ==
  data: theta input; zero_phase_detect input; trig_sig output; hThetaLast data_store_memory; lag_val input; hZeroPhaseDetectLast data_store_memory; hZeroPhaseFlag data_store_memory
function trig_sig = PhaseLag(theta, zero_phase_detect, lag_val)
global hZeroPhaseDetectLast;
global hZeroPhaseFlag;

if (zero_phase_detect > 0) && (hZeroPhaseDetectLast == 0)
    % rising-edge detection
    hZeroPhaseFlag = 1;
end

if (hZeroPhaseFlag == 1) && (theta <= lag_val)
    % wait for theta increasing
    phase_lag_trig = 0;
elseif (hZeroPhaseFlag == 1) && (theta > lag_val)
    phase_lag_trig = 1;
    hZeroPhaseFlag = 0; % reset zero_phase_detection event
else
    phase_lag_trig = 0;
end

hZeroPhaseDetectLast = zero_phase_detect;

trig_sig = phase_lag_trig;

== matlab function auto_sync_scan_module/Auto Sync Scan Module (Voltage)/CoreFunction ==
  data: InStartFlag input; PhaseLockSig input; FreqSeq input; OutUa output; InjectAmp input; InjectMode input; t_disturb input; t_rec input; t_rest input; OutUb output; OutUc output; OutClock output; OutDisturbFlag output; OutRecFlag output; OutRestFlag output; OutFreqIndex output; OutFreqNowScan output; OutStatus output; OutPosOrNegFlag output; hStepCounter data_store_memory; hFreqIndex data_store_memory; hStartFlagMem data_store_memory; hPhaseLockFlag data_store_memory; SampleTimeInput input; hRisingEdgeGot data_store_memory
function [OutUa, OutUb, OutUc, ...
    OutClock, OutDisturbFlag, OutRecFlag, OutRestFlag, ...
    OutFreqIndex, OutFreqNowScan, OutStatus, OutPosOrNegFlag] = ...
    fcn(InStartFlag, PhaseLockSig, FreqSeq, InjectAmp, InjectMode, ...
    t_disturb, t_rec, t_rest, SampleTimeInput)
% InjectMode = 1, Positive sequence
% InjectMode = 2, Negative sequence
% InjectMode = 3, Positive et Negative simutaneously

global hStepCounter;
global hFreqIndex; 
global hStartFlagMem;
global hPhaseLockFlag;
global hRisingEdgeGot; % record a rising-edge get event, cleared untile all frequency are scanned.

this_freq = 0; %% only used for output
FreqSeqLength = length(FreqSeq);

SAMPLE_TIME = SampleTimeInput;
SAMPLE_FREQ = 1/SAMPLE_TIME;

T_DISTURB	= t_disturb * SAMPLE_FREQ;
T_REC 		= t_rec * SAMPLE_FREQ;
T_REST 		= t_rest * SAMPLE_FREQ;

clock_t		= 0;
start_flag	= 0;
status_code	= 0;
ua			= 0; 
ub			= 0; 
uc			= 0;
omega		= 0;
disturb_flag = 0;
rec_flag    = 0;
rest_flag   = 0;

if hPhaseLockFlag == 0 && PhaseLockSig == 1  % Phase-lock event catch, reset by every scan step
    hPhaseLockFlag = 1;
end


start_flag = InStartFlag;
if (start_flag >= 1 && hStartFlagMem == 0) % rising-edge event catch
	hRisingEdgeGot = 1;
	hFreqIndex = 1;
end

if (start_flag >= 1 && hRisingEdgeGot == 1) % once triggerd, loop until all frequences are scanned
	if (hFreqIndex >=1 && hFreqIndex <= FreqSeqLength && hPhaseLockFlag == 1)
		status_code = 1;
		if (hStepCounter <= (T_DISTURB - T_REC))
			disturb_flag = 1;
			rec_flag = 0;
			rest_flag = 0;
			hStepCounter = hStepCounter + 1;
        elseif ((hStepCounter > (T_DISTURB - T_REC)) && (hStepCounter <= T_DISTURB) && hPhaseLockFlag == 1)
			disturb_flag = 1;
			rec_flag = 1;
			rest_flag = 0;
			hStepCounter = hStepCounter + 1;
        elseif ((hStepCounter > T_DISTURB) && hStepCounter <= (T_DISTURB + T_REST) && hPhaseLockFlag == 1)
			disturb_flag = 0;
			rec_flag = 0;
			rest_flag = 1;
			hStepCounter = hStepCounter + 1;
        else
			hStepCounter = int32(0);
			hFreqIndex = hFreqIndex + 1;
			ua = 0; ub = 0; uc = 0;
            hPhaseLockFlag = 0;
        end

		if (disturb_flag == 1) 
            this_freq = FreqSeq(hFreqIndex); % only used for output port 
			clock_t = double(hStepCounter) * SAMPLE_TIME;
			omega = 2.0 * FreqSeq(hFreqIndex) * pi;
            
			if (InjectMode == 1)
				ua = InjectAmp * sin(omega * clock_t);
				ub = InjectAmp * sin(omega * clock_t - 2.0*pi/3.0);
				uc = InjectAmp * sin(omega * clock_t + 2.0*pi/3.0);
			
            elseif (InjectMode == 2)
				ua = InjectAmp * sin(omega * clock_t);
				ub = InjectAmp * sin(omega * clock_t + 2.0*pi/3.0);
				uc = InjectAmp * sin(omega * clock_t - 2.0*pi/3.0);
                
            elseif (InjectMode == 3)
                ua = InjectAmp * sin(omega * clock_t);
				ub = 0.5 * InjectAmp * sin(omega * clock_t + 2.0*pi/3.0) + ...
                     0.5 * InjectAmp * sin(omega * clock_t - 2.0*pi/3.0);
				uc = ub;
            else
                % other InjectMode to be write here.
            end
        end
	elseif hFreqIndex > FreqSeqLength
		status_code = 2;
		hRisingEdgeGot = 0;
		ua = 0; ub = 0; uc = 0;
	else
		ua = 0; ub = 0; uc = 0;
		status_code = 3;
	end

else % start_flag == 0 || hRisingEdgeGot == 0

	hFreqIndex = 1;

	status_code = 0;
	disturb_flag = 0;
	rec_flag = 0;
	rest_flag = 0;
	hStepCounter = int32(0);
	clock_t = double(hStepCounter) * SAMPLE_TIME;
	ua = 0; ub = 0; uc = 0;
end
	hStartFlagMem = int32(start_flag);  % record start_flag
	OutUa = ua;
	OutUb = ub;
	OutUc = uc;

	OutStatus = status_code;
	OutFreqIndex = hFreqIndex;
	OutFreqNowScan = this_freq;
	OutClock = clock_t;
	OutDisturbFlag = disturb_flag;
	OutRecFlag = rec_flag;
	OutRestFlag = rest_flag;
    OutPosOrNegFlag = InjectMode;
end

== matlab function auto_sync_scan_module/Auto Sync Scan Module (Voltage)/PhaseLag ==
  data: theta input; zero_phase_detect input; trig_sig output; hThetaLast data_store_memory; lag_val input; hZeroPhaseDetectLast data_store_memory; hZeroPhaseFlag data_store_memory
function trig_sig = PhaseLag(theta, zero_phase_detect, lag_val)
global hZeroPhaseDetectLast;
global hZeroPhaseFlag;

if (zero_phase_detect > 0) && (hZeroPhaseDetectLast == 0)
    % rising-edge detection
    hZeroPhaseFlag = 1;
end

if (hZeroPhaseFlag == 1) && (theta <= lag_val)
    % wait for theta increasing
    phase_lag_trig = 0;
elseif (hZeroPhaseFlag == 1) && (theta > lag_val)
    phase_lag_trig = 1;
    hZeroPhaseFlag = 0; % reset zero_phase_detection event
else
    phase_lag_trig = 0;
end

hZeroPhaseDetectLast = zero_phase_detect;

trig_sig = phase_lag_trig;

== matlab function auto_sync_scan_module/Auto Sync Scan Module (Voltage)/ZeroPhaseDetect ==
  data: theta input; y output; hThetaLast data_store_memory
function y = ZeroPhaseDetect(theta)
global hThetaLast;


if theta < hThetaLast
    zero_phase_detect = 1;
else
    zero_phase_detect = 0;
end
hThetaLast = theta;

y = zero_phase_detect;
